simulink model "TSMC2"  (R2026b)
settings: Solver=ode4  StopTime=20  FixedStep=1e-3
settings Model: Creator=Yahoff  LastModifiedBy=Yahoff

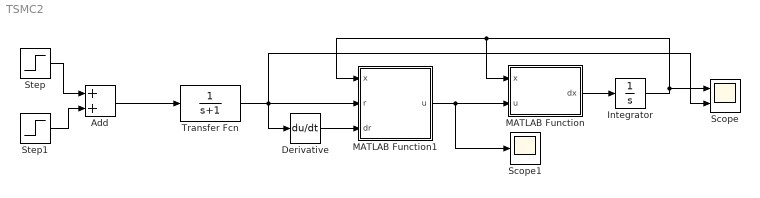
== system TSMC2 ==
  Add : Sum
  Derivative : Derivative
  Integrator : Integrator  InitialCondition=[1;-1]
  MATLAB Function : MATLAB Function  TreatAsAtomicUnit=on
  MATLAB Function1 : MATLAB Function  TreatAsAtomicUnit=on
  Scope : Scope  NumInputPorts=2
      settings: ActiveDisplayYMinimum=-2.3171090595239825  ActiveDisplayYMaximum=3.5912390259061104
  Scope1 : Scope
      settings: ActiveDisplayYMinimum=-13.250531460184636  ActiveDisplayYMaximum=17.63187581376409
  Step : Step  FinalValue=2  SampleTime=0
  Step1 : Step  Time=10  SampleTime=0
  Transfer Fcn : TransferFcn  Denominator=[1 1]
  wires:
  MATLAB Function/1(dx) -> Integrator/1
  Integrator/1 -> Scope/1, MATLAB Function/1(x), MATLAB Function1/1(x)
  MATLAB Function1/1(u) -> Scope1/1, MATLAB Function/2(u)
  Add/1 -> Transfer Fcn/1
  Transfer Fcn/1 -> Derivative/1, Scope/2, MATLAB Function1/2(r)
  Derivative/1 -> MATLAB Function1/3(dr)
  Step/1 -> Add/1
  Step1/1 -> Add/2

== matlab function TSMC2/MATLAB Function ==
  data: x input size=2; u input; dx output size=2
function dx  = fcn(x,u)

x1 = x(1);
x2 = x(2);

dx1 = x2;
dx2 = sin(x1+x2)*cos(x1*x2)+u;

dx = [dx1;dx2];

== matlab function TSMC2/MATLAB Function1 ==
  data: x input; u output; r input; dr input
function u = fcn(x,r,dr)

ga    = 1;
K     = 10;
m     = 2;

x1 = x(1);
x2 = x(2);

e1 =  r-x1;
e2 = dr-x2;

st = e1+ (1/m)*sigpow(e2,ga);
u = (m/ga)*sigpow(e2,2-ga)+K*sign(st);

function v = sigpow(x,p)
    if x>0
        v = abs(x)^p;
    else if x<0   
        v = -abs(x)^p;
    else
        v = 0;
    end
end
